simulink model "lab6_task4_model2"  (R2024b)
settings: Solver=ode45  StartTime=0.0  StopTime=10.0  MaxStep=0.01  RelTol=1e-3
settings Model: Creator=Beanie  LastModifiedBy=Beanie

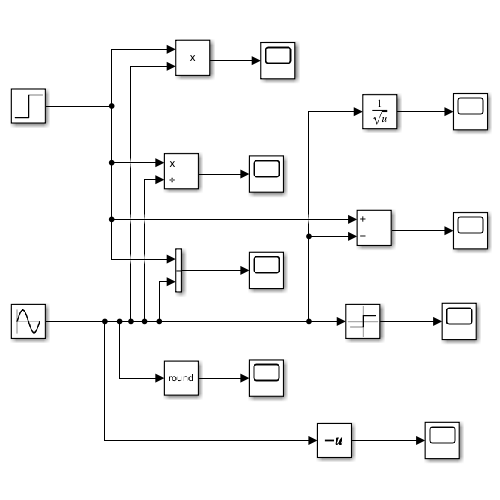
[thumbnail: Simulink's stored preview of the top-level diagram]
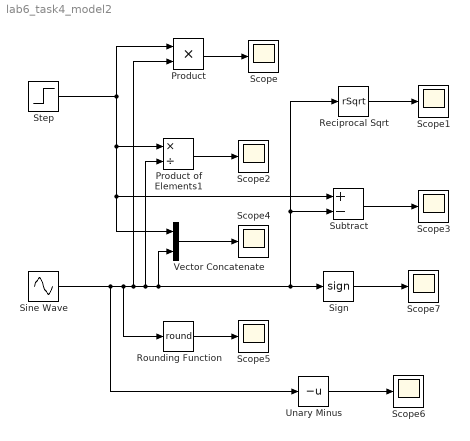
== system lab6_task4_model2 ==
  Product : Product
  Product of Elements1 : Product  Inputs=*/
  Reciprocal Sqrt : Sqrt  Operator=rSqrt
  Rounding Function : Rounding  Operator=round
  Scope{,1..7} (8 alike) : Scope
  Sign : Signum
  Sine Wave : Sin  Frequency=2*pi  SampleTime=0
  Step : Step  SampleTime=0
  Subtract : Sum  Inputs=+-
  Unary Minus : UnaryMinus
  Vector Concatenate : Concatenate
  wires:
  Vector Concatenate/1 -> Scope4/1
  Rounding Function/1 -> Scope5/1
  Unary Minus/1 -> Scope6/1
  Sign/1 -> Scope7/1
  Subtract/1 -> Scope3/1
  Reciprocal Sqrt/1 -> Scope1/1
  Product/1 -> Scope/1
  Product of Elements1/1 -> Scope2/1
  Step/1 -> Vector Concatenate/1, Subtract/1, Product of Elements1/1, Product/1
  Sine Wave/1 -> Unary Minus/1, Rounding Function/1, Product/2, Product of Elements1/2, Vector Concatenate/2, Reciprocal Sqrt/1, Subtract/2, Sign/1
